simulink model "pv20kanfis"  (R2016a)
settings: Solver=ode23s  StartTime=0.0  StopTime=4  MaxStep=0.0001
undefined symbols (not defined in the file or in its folder): sigbuilder_block
libraries: powerlib x9, powerlib_extras x2, fuzblock x1, re_lib x1, powerlib_meascontrol x1
settings Model: Creator=venka  LastModifiedBy=CHANDRA
settings SolverCC: ZeroCrossControl=DisableAll  AlgebraicLoopSolver=LineSearch
settings DataIOCC: LimitDataPoints=on  MaxDataPoints=10000
settings DebuggingCC: AllowSymbolicDim=off
settings ConfigComp: CovSFcnEnable=off
settings SimscapeCC: SimscapeLogType=all  SimscapeLogDataHistory=10000

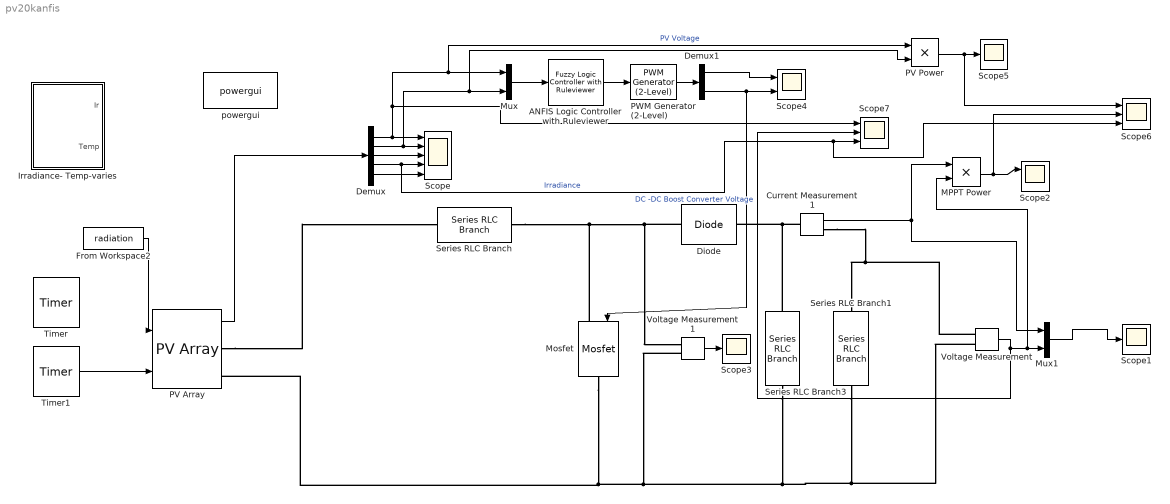
== system pv20kanfis ==
  ANFIS Logic Controller with Ruleviewer : fuzblock/Fuzzy Logic  Controller  with Ruleviewer  fismatrix=ap  Ts=0.06
  Current Measurement1 : powerlib/Measurements/Current Measurement  PhasorSimulation=off  OutputType=Complex  PSBequivalent=0
  Demux : Demux  Outputs=5
  Demux1 : Demux  Outputs=2
  Diode : powerlib/Power Electronics/Diode  Ron=0.5  Lon=0  Vf=0.8  IC=0  UseSnubber=off  Rs=1e5  Cs=250e-9  Measurements=off
  From Workspace2 : FromWorkspace  VariableName=radiation  SampleTime=0
  Irradiance- Temp-varies : Subsystem  Tag=STV Subsys  LoadFcn=sigbuilder_block('load');  StartFcn=sigbuilder_block('start');  StopFcn=sigbuilder_block('stop');  ClipboardFcn=sigbuilder_block('clipboard');  mask(Sigbuilder block){}
      mask help: Sigbuilder GUI
      mask init:
      | if ~strcmp(get_param(bdroot(gcbh),'SimulationStatus'),'stopped') tuvar = sigbuilder_block('maskInit'); end
      settings: CopyFcn=sigbuilder_block('copy');  DeleteFcn=sigbuilder_block('delete');  ModelCloseFcn=sigbuilder_block('modelClose');  PreSaveFcn=sigbuilder_block('preSave');  PauseFcn=sigbuilder_block('pause')  ContinueFcn=sigbuilder_block('continue')  NameChangeFcn=sigbuilder_block('namechange');  OpenFcn=sigbuilder_block('open',[6 30 1012.5 447.75 ]);  CloseFcn=sigbuilder_block('close');
      mask Display: plot(0, 0, 100, 100,[2, 2, 32, 32, 2], [68, 8, 8, 68, 68],[32, 2], [38, 38], [32, 19, 2],[53, 60, 44], [32, 17, 17, 2],[16, 16, 31, 31]);txt = getActiveGroup(gcbh);text(2, 100, txt,'verticalAlignment', 'top');
  MPPT Power : Product
  Mosfet : powerlib/Power Electronics/Mosfet  Ron=0.1  Lon=0  Rd=0.01  Vfd=0.8  IC=0  Rs=1e5  Cs=inf  Measurements=off
  Mux : Mux  Inputs=2
  Mux1 : Mux  Inputs=2
  PV Array : re_lib/Solar/PV Array  Npar=10  Nser=10  PlotType=array @ 1000 W/m2 & specified temperatures  S_vec="[ 1000  500  100 ]"  Temp_C_vec="[ 45 25  ]"  ModuleName=1Soltech 1STH-215-P  PlotWhenSelected=off  Pm=213.15  Ncell=60  Voc=36.3  Isc=7.84  Vm=29  Im=7.35  beta_Voc_pc=-0.36099  alpha_Isc_pc=0.102  beta_Voc=-0.13104  alpha_Isc=0.007997  IL=7.8649  I0=2.9259e-10  nI=0.98117  Rsh=313.3991  Rs=0.39383  BAL=off  Tc=1e-6  Tfilter=5e-5
  PV Power : Product
  PWM Generator (2-Level) : powerlib_meascontrol/Pulse & Signal Generators/PWM Generator (2-Level)  ModulatorType=Single-phase half-bridge (2 pulses)  ModulatorMode=Unsynchronized  Fc=1500  Pc=0  nF=27  MinMax="[ 0  1 ]"  SamplingTechnique=Natural  ModulatingSignals=off  m=0.8  Freq=60  Phase=0  Ts=0  ShowCarrierOutport=off
  Scope : Scope  NumInputPorts=5
  Scope1 : Scope
  Scope2 : Scope  NumInputPorts=2
  Scope3 : Scope
  Scope4 : Scope  NumInputPorts=2
  Scope5 : Scope
  Scope6 : Scope  NumInputPorts=3
  Scope7 : Scope  NumInputPorts=3
  Series RLC Branch : powerlib/Elements/Series RLC Branch  LConnTagsString=__new0  RConnTagsString=__new0  BranchType=L  Resistance=0.001  Inductance=0.05  SetiL0=off  InitialCurrent=0  Capacitance=1e-6  Setx0=off  InitialVoltage=0  Measurements=None
  Series RLC Branch1 : powerlib/Elements/Series RLC Branch  LConnTagsString=__new0  RConnTagsString=__new0  BranchType=R  Resistance=14  Inductance=0.1  SetiL0=off  InitialCurrent=0  Capacitance=100e-6  Setx0=off  InitialVoltage=0  Measurements=None
  Series RLC Branch3 : powerlib/Elements/Series RLC Branch  LConnTagsString=__new0  RConnTagsString=__new0  BranchType=C  Resistance=6  Inductance=0.1  SetiL0=off  InitialCurrent=0  Capacitance=100e-6  Setx0=off  InitialVoltage=0  Measurements=None
  Timer : powerlib_extras/Control  Blocks/Timer  t=[0 1 2 3 4]  e=[0.25 0.5 0.75 1 0.25]*1e3
  Timer1 : powerlib_extras/Control  Blocks/Timer  t=[0 1 2 3 4]  e=[25 30 35 25 25]
  Voltage Measurement : powerlib/Measurements/Voltage Measurement  PhasorSimulation=off  OutputType=Complex  PSBequivalent=0
  Voltage Measurement1 : powerlib/Measurements/Voltage Measurement  PhasorSimulation=off  OutputType=Complex  PSBequivalent=0
  powergui : powerlib/powergui  Priority=1  SimulationMode=Discrete  SolverType=Tustin/Backward Euler (TBE)  SampleTime=1e-3  frequency=60  SPID=on  DisableSnubberDevices=off  DisableRonSwitches=off  DisableVfSwitches=off  SwTol=0  DisplayEquations=off  Interpol=off  ExternalGateDelay=off  methode=off  Ts=100  FunctionMessages=off  echomessages=off  HookPort=off  EnableUseOfTLC=off  x0status=blocks  frequencyindice=0  Pbase=100e6  ErrMax=1e-4  Iterations=50  UnitsV=kV  UnitsW=MW  buscounter=0  RestoreLinks=warning  ResistiveCurrentMeasurement=off  Frange=[0:2:500]  Ylog=off  Xlog=on  ShowGrid=off  save=off  variable=ZData  structure=0  ZoomFFT=off  StartTime=0.0  cycles=1  DisplayStyle=1  fundamental=60  FreqAxis=off  MaxFrequency=1000  frequencyindicesteady=1  RmsSteady=1  display=off
  wires:
  PV Array/1 -> Demux/1
  Voltage Measurement/1 -> Scope7/2, MPPT Power/2, Mux1/2  "DC -DC Boost Converter Voltage"
  Mux1/1 -> Scope1/1
  Demux/1 -> Scope7/1, PV Power/1, Mux/1, Scope/1  "PV Voltage"
  Demux/2 -> PV Power/2, Mux/2, Scope/2
  Demux/3 -> Scope/3
  Demux/4 -> Scope6/3, Scope7/3, Scope/4  "Irradiance"
  Demux/5 -> Scope/5
  Mux/1 -> ANFIS Logic Controller with Ruleviewer/1
  ANFIS Logic Controller with Ruleviewer/1 -> PWM Generator (2-Level)/1
  MPPT Power/1 -> Scope6/2, Scope2/1
  Voltage Measurement1/1 -> Scope3/1
  Current Measurement1/1 -> MPPT Power/1, Mux1/1
  PWM Generator (2-Level)/1 -> Demux1/1
  Demux1/1 -> Scope4/1
  Demux1/2 -> Mosfet/1, Scope4/2
  PV Power/1 -> Scope6/1, Scope5/1
  ? -> Scope2/2
  From Workspace2/1 -> PV Array/1
  Timer1/1 -> PV Array/2
  connections:
  Series RLC Branch/RConn1 -- Mosfet/LConn1 -- Diode/LConn1 -- Voltage Measurement1/LConn1
  PV Array/RConn2 -- Mosfet/RConn1 -- Voltage Measurement/LConn2 -- Series RLC Branch1/RConn1 -- Series RLC Branch3/RConn1 -- Voltage Measurement1/LConn2
  Current Measurement1/LConn1 -- Series RLC Branch3/LConn1 -- Diode/RConn1
  Current Measurement1/RConn1 -- Voltage Measurement/LConn1 -- Series RLC Branch1/LConn1
  PV Array/RConn1 -- Series RLC Branch/LConn1

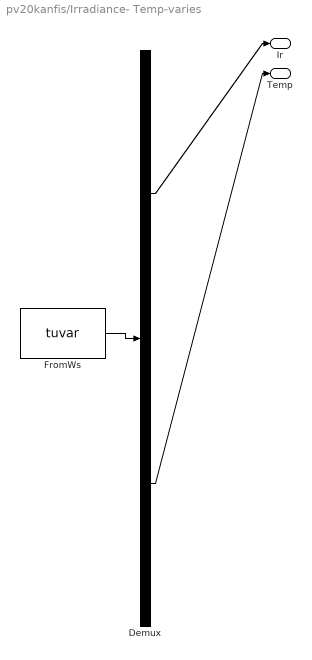
== system pv20kanfis/Irradiance- Temp-varies ==
  Demux : Demux  Tag=STV Demux  Outputs=2
  FromWs : FromWorkspace  Tag=STV FromWs  VariableName=tuvar  SampleTime=0
      SigBuilderData=|
      | common.afterFinalStr = 'Extrapolate'
      | common.sampleTime = '0'
      | dataSet(1).timeRange = [0 1]
      | dataSet(1).name = 'Constant Irradiance'
      | dataSet(2).timeRange = [0 1]
      | dataSet(2).name = 'Step Irradiance'
      | dataSet(3).timeRange = [0 3]
      | dataSet(3).name = 'Ramp-up/down Irradiance'
      | sbobj.Groups(1).Name = 'Constant Irradiance'
      | sbobj.Groups(1).Signals(1).Name = 'Ir'
      | sbobj.Groups(1).Signals(1).XData = [0 1]
      | sbobj.Groups(1).Signals(1).YData = [1000 1000]
      | sbobj.Groups(1).Signals(2).Name = 'Temp'
      | sbobj.Groups(1).Signals(2).XData = [0 1 1 2]
      | sbobj.Groups(1).Signals(2).YData = [0 0 1 1]
      | sbobj.Groups(1).TimeRange = [0 1]
      | sbobj.Groups(2).Name = 'Step Irradiance'
      | sbobj.Groups(2).Signals(1).Name = 'Ir'
      | sbobj.Groups(2).Signals(1).XData = [0 0.252 0.252 1]
      | sbobj.Groups(2).Signals(1).YData = [600 600 1000 1000]
      | sbobj.Groups(2).Signals(2).Name = 'Temp'
      | sbobj.Groups(2).Signals(2).XData = [0 1 1 2]
      | sbobj.Groups(2).Signals(2).YData = [0 0 1 1]
      | sbobj.Groups(2).TimeRange = [0 1]
      | sbobj.Groups(3).Name = 'Ramp-up/down Irradiance'
      | sbobj.Groups(3).Signals(1).Name = 'Ir'
      | sbobj.Groups(3).Signals(1).XData = [0 0.6 1.1 1.2 1.7 3]
      | sbobj.Groups(3).Signals(1).YData = [1000 1000 250 250 1000 1000]
      | sbobj.Groups(3).Signals(2).Name = 'Temp'
      | sbobj.Groups(3).Signals(2).XData = [0 2 2.1 3]
      | sbobj.Groups(3).Signals(2).YData = [25 25 50 50]
      | sbobj.Groups(3).TimeRange = [0 3]
  Ir : Outport  Tag=STV Outport
  Temp : Outport  Tag=STV Outport  Port=2
  wires:
  Demux/2 -> Temp/1
  FromWs/1 -> Demux/1
  Demux/1 -> Ir/1
